simulink model "elsistema"  (R2020b)
settings: Solver=ode15s  StartTime=0.0  StopTime=10  MaxStep=1E-2  RelTol=1e-3
libraries: fl_lib x12, nesl_utility x8, ee_lib x2, pid_lib x1
settings Model: Creator=MSI  LastModifiedBy=hiram
settings SolverCC: AlgebraicLoopSolver=LineSearch
settings DataIOCC: SaveOutput=off  SignalLogging=off  DSMLogging=off  ReturnWorkspaceOutputs=off  TimeSaveName=t
settings DebuggingCC: AlgebraicLoopMsg=none  ArtificialAlgebraicLoopMsg=none  MaxConsecutiveZCsMsg=none  UnconnectedInputMsg=none  UnconnectedOutputMsg=none  UnconnectedLineMsg=none  ModelReferenceExtraNoncontSigs=none  OperatingPointInterfaceChecksumMismatchMsg=none
settings ModelReferenceCC: EnableRefExpFcnMdlSchedulingChecks=off

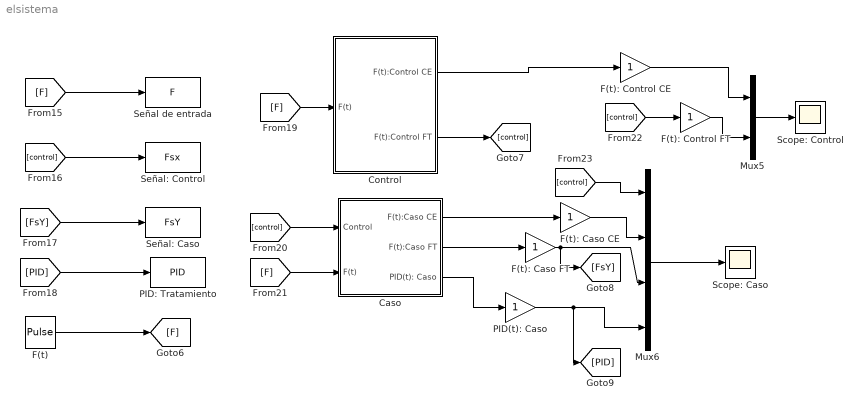
== system elsistema ==
  Caso : Subsystem
  Control : Subsystem
  F(t) : DiscretePulseGenerator  PulseType=Time based  Period=10  PulseWidth=10  PhaseDelay=1
  F(t): Caso CE : Gain
  F(t): Caso FT : Gain
  F(t): Control CE : Gain
  F(t): Control FT : Gain
  Mux5 : Mux  Inputs=2
  Mux6 : Mux
  PID(t): Caso : Gain
  PID: Tratamiento : ToWorkspace  VariableName=PID  SampleTime=-1
  Scope: Caso : Scope
  Scope: Control : Scope
  Señal de entrada : ToWorkspace  VariableName=F  SampleTime=-1
  Señal: Caso : ToWorkspace  VariableName=FsY  SampleTime=-1
  Señal: Control : ToWorkspace  VariableName=Fsx  SampleTime=-1
  wires:
  [F] -> Señal de entrada/1
  [control] -> Señal: Control/1
  [FsY] -> Señal: Caso/1
  [PID] -> PID: Tratamiento/1
  F(t)/1 -> [F]
  [F] -> Control/1(F(t))
  [control] -> Caso/1(Control)
  [F] -> Caso/2(F(t))
  Control/2(F(t):Control FT) -> [control]
  F(t): Control CE/1 -> Mux5/1
  [control] -> F(t): Control FT/1
  F(t): Control FT/1 -> Mux5/2
  Mux5/1 -> Scope: Control/1
  Caso/1(F(t):Caso CE) -> F(t): Caso CE/1
  F(t): Caso CE/1 -> Mux6/2
  [control] -> Mux6/1
  Caso/2(F(t):Caso FT) -> F(t): Caso FT/1
  F(t): Caso FT/1 -> Mux6/3, [FsY]
  PID(t): Caso/1 -> [PID], Mux6/4
  Caso/3(PID(t): Caso) -> PID(t): Caso/1
  Mux6/1 -> Scope: Caso/1
  Control/1(F(t):Control CE) -> F(t): Control CE/1

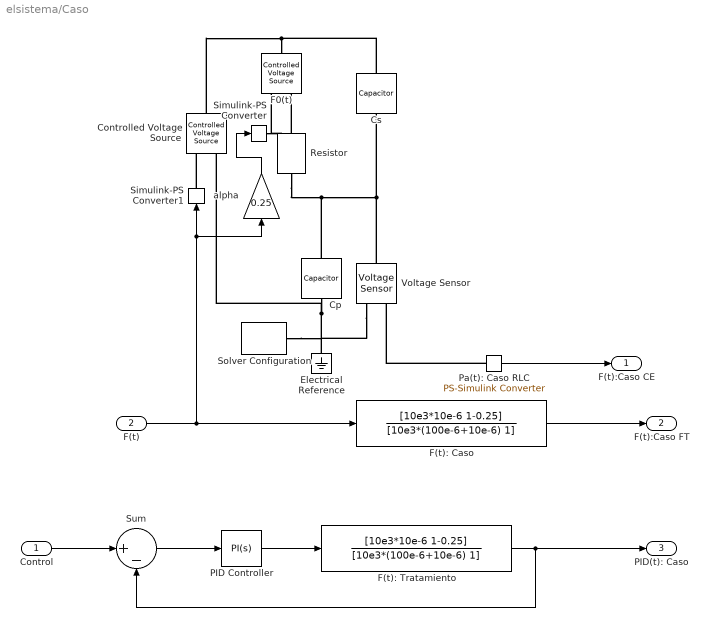
== system elsistema/Caso ==
  Control : Inport
  F(t) : Inport  Port=2
  Controlled Voltage Source : fl_lib/Electrical/Electrical Sources/Controlled Voltage Source
  Cp : fl_lib/Electrical/Electrical Elements/Capacitor  c=1e-6 F  r=1e-6 Ohm  g=0 1/Ohm  i_specify=off  i_priority=None  i=0 A  i_nominal_specify=off  i_nominal_unit=A  i_nominal_value=1  v_specify=off  v_priority=None  v=0 V  v_nominal_specify=off  v_nominal_unit=V  v_nominal_value=1  vc_specify=off  vc_priority=High  vc=0 V  vc_nominal_specify=off  vc_nominal_unit=V  vc_nominal_value=1
  Cs : fl_lib/Electrical/Electrical Elements/Capacitor  c=1e-6 F  r=1e-6 Ohm  g=0 1/Ohm  i_specify=off  i_priority=None  i=0 A  i_nominal_specify=off  i_nominal_unit=A  i_nominal_value=1  v_specify=off  v_priority=None  v=0 V  v_nominal_specify=off  v_nominal_unit=V  v_nominal_value=1  vc_specify=off  vc_priority=High  vc=0 V  vc_nominal_specify=off  vc_nominal_unit=V  vc_nominal_value=1
  Electrical Reference : fl_lib/Electrical/Electrical Elements/Electrical Reference
  F(t): Caso : TransferFcn  Numerator=[10e3*10e-6 1-0.25]  Denominator=[10e3*(100e-6+10e-6) 1]
  F(t): Tratamiento : TransferFcn  Numerator=[10e3*10e-6 1-0.25]  Denominator=[10e3*(100e-6+10e-6) 1]
  F0(t) : fl_lib/Electrical/Electrical Sources/Controlled Voltage Source
  PID Controller : pid_lib/PID Controller  Controller=PI  Form=Parallel  TimeDomain=Continuous-time  UseExternalTs=off  SampleTime=-1  IntegratorMethod=Forward Euler  FilterMethod=Forward Euler  ControllerParametersSource=internal  P=0.21161  I=3765.3621  D=0  UseFilter=on  N=100  TunerSelectOption=Transfer Function Based (PID Tuner App)  InitialConditionSource=internal  InitialConditionForIntegrator=0  InitialConditionForFilter=0  DifferentiatorICPrevScaledInput=0  ExternalReset=none  TrackingMode=off  Kt=1  LimitOutput=off  SatLimitsSource=internal  UpperSaturationLimit=inf  LowerSaturationLimit=-inf  LinearizeAsGain=on  AntiWindupMode=none  Kb=1  POutMin=[]  POutMax=[]  IOutMin=[]  IOutMax=[]  DOutMin=[]  DOutMax=[]  NOutMin=[]  NOutMax=[]  SumOutMin=[]  SumOutMax=[]  SaturationOutMin=[]  SaturationOutMax=[]  PParamMin=[]  PParamMax=[]  IParamMin=[]  IParamMax=[]  DParamMin=[]  DParamMax=[]  NParamMin=[]  NParamMax=[]  KbParamMin=[]  KbParamMax=[]  KtParamMin=[]  KtParamMax=[]  KbOutMin=[]  KbOutMax=[]  KtOutMin=[]  KtOutMax=[]  IntegratorOutMin=[]  IntegratorOutMax=[]  FilterOutMin=[]  FilterOutMax=[]  SumI1OutMin=[]  SumI1OutMax=[]  SumI2OutMin=[]  SumI2OutMax=[]  SumI3OutMin=[]  SumI3OutMax=[]  SumI4OutMin=[]  SumI4OutMax=[]  SumDOutMin=[]  SumDOutMax=[]  DifferentiatorOutMin=[]  DifferentiatorOutMax=[]  FilterDiffOutCoefMin=[]  FilterDiffOutCoefMax=[]  ReciprocalOutMin=[]  ReciprocalOutMax=[]  SumDenOutMin=[]  SumDenOutMax=[]  SumNumOutMin=[]  SumNumOutMax=[]  DivideOutMin=[]  DivideOutMax=[]  UdiffTsProdOutMin=[]  UdiffTsProdOutMax=[]  NTsProdOutMin=[]  NTsProdOutMax=[]  UintegralTsProdOutMin=[]  UintegralTsProdOutMax=[]  UngainTsProdOutMin=[]  UngainTsProdOutMax=[]  IntegratorContinuousStateAttributes=''  IntegratorStateMustResolveToSignalObject=off  IntegratorRTWStateStorageClass=Auto  FilterContinuousStateAttributes=''  FilterStateMustResolveToSignalObject=off  FilterRTWStateStorageClass=Auto  ParallelPVariant=InternalParameters  IdealPVariant=Disabled  IVariant=InternalParameters  DVariant=Disabled  IntegratorVariant=Continuous  SatVariant=Disabled  AWVariant=Passthrough  PCopyVariant=Disabled  TRVariant=Disabled  FdbkBlocksVariant=Forward  IdealPFdbkVariant=Disabled  SatFdbkVariant=Disabled  DerivativeFilterVariant=Disabled  NVariant=Disabled  NCopyVariant=Disabled_SignalSpec  FilterICVariant=Disabled  IntegratorICVariant=InternalICs  ExternalResetVariant=Disabled  TRSumVariant=Passthrough  SumFdbkVariant=Disabled  SumVariant=Sum_PI  TsampFilterVariant=InternalTs  TsampNgainVariant=Passthrough  TsampIntegralVariant=Passthrough  ExternalSaturationOutDataTypeStr=Inherit: Same as second input
  Pa(t): Caso RLC : nesl_utility/PS-Simulink Converter  PhysicalDomain=network_engine_domain  SubClassName=ps_output  LeftPortType=input  RightPortType=output  PseudoPeriodic=off  Frequencies=[]  Unit=inherit  AffineConversion=off
  Resistor : ee_lib/Passive/Resistor  R=1 Ohm  R_tol=5  enable_R_tol=0  tol_distribution=1  nSigma=4  enable_operating_limits=0  operating_limit_action=2  max_working_voltage=100 V  power_rating=1 W  enable_faults=0  fault_action=1  R_faulted=inf Ohm  enable_temporal_fault=0  t_fault=1 s  enable_behavioral_fault=0  max_permissible_current=1 A  t_fail_on_current=1 s  noise_mode=0  sample_time=1e-3 s  repeatability=1  auto_seed=3499211588  user_seed=0  Tdevice=25 degC  alpha=3.93e-3 1/K  Tmeas=25 degC  thermal_mass=100 J/K  power_derating_T1=70 degC  power_derating_T2=155 degC  operating_temperature_range_vec=[-50, 150] degC  temperature_specify=off  temperature_priority=High  temperature=298.15 K  temperature_nominal_specify=off  temperature_nominal_unit=K  temperature_nominal_value=1
  Simulink-PS Converter : nesl_utility/Simulink-PS Converter  PhysicalDomain=network_engine_domain  SubClassName=ps_input  LeftPortType=input  RightPortType=output  PseudoPeriodic=off  Frequencies=[]  NoiseDistribution=none  NoiseParameters=[]  Unit=1  AffineConversion=off  FilteringAndDerivatives=provide  SimscapeFilterOrder=1  InputFilterTimeConstant=0.001  UdotUserProvided=0
  Simulink-PS Converter1 : nesl_utility/Simulink-PS Converter  PhysicalDomain=network_engine_domain  SubClassName=ps_input  LeftPortType=input  RightPortType=output  PseudoPeriodic=off  Frequencies=[]  NoiseDistribution=none  NoiseParameters=[]  Unit=1  AffineConversion=off  FilteringAndDerivatives=provide  SimscapeFilterOrder=1  InputFilterTimeConstant=0.001  UdotUserProvided=0
  Solver Configuration : nesl_utility/Solver Configuration  PhysicalDomain=network_engine_domain  SubClassName=solver  LeftPortType=input  RightPortType=generic  Tones=[]  Harmonics=[]  SimulateNoise=off  Profile=off  UseLocalSampling=off  EnableSwitchedLinearOptims=on  FrequencyDomain=off  UseCCode=off  RelTol=0.001  AbsTol=1e-06  MinStep=1e-09  ToWorkspace=off  RevertToSquareIcSolve=off  NumHomotopyIterations=100  PhasorMode=off  PhasorModeNumHarmonics=1  DoDC=off  ResidualTolerance=1e-09  UseLocalSolver=off  LocalSolverChoice=NE_BACKWARD_EULER_ADVANCER  LocalSolverSampleTime=0.001  DoFixedCost=off  MaxNonlinIter=3  MaxModeIter=2  ComputeImpulses=off  ImpulseIterations=2  LinearAlgebra=auto  EquationFormulation=NE_TIME_EF  DelaysMemoryBudget=1024  AutomaticFiltering=on  FilteringTimeConstant=0.001  PartitionStorageMethod=AS_NEEDED  PartitionMemoryBudget=1024  PartitionMethod=ROBUST
  Sum : Sum  Inputs=|+-
  Voltage Sensor : fl_lib/Electrical/Electrical Sensors/Voltage Sensor
  alpha : Gain  Gain=0.25
  F(t):Caso CE : Outport
  F(t):Caso FT : Outport  Port=2
  PID(t): Caso : Outport  Port=3
  wires:
  alpha/1 -> Simulink-PS Converter/1
  F(t)/1 -> F(t): Caso/1, alpha/1, Simulink-PS Converter1/1
  Pa(t): Caso RLC/1 -> F(t):Caso CE/1
  F(t): Caso/1 -> F(t):Caso FT/1
  Control/1 -> Sum/1
  Sum/1 -> PID Controller/1
  PID Controller/1 -> F(t): Tratamiento/1
  F(t): Tratamiento/1 -> Sum/2, PID(t): Caso/1
  connections:
  Controlled Voltage Source/LConn1 -- Cs/LConn1 -- F0(t)/LConn1
  Resistor/LConn1 -- F0(t)/RConn2
  Resistor/RConn1 -- Cp/LConn1 -- Cs/RConn1 -- Voltage Sensor/LConn1
  Cp/RConn1 -- Solver Configuration/RConn1 -- Voltage Sensor/RConn2 -- Electrical Reference/LConn1 -- Controlled Voltage Source/RConn2
  Simulink-PS Converter/RConn1 -- F0(t)/RConn1
  Simulink-PS Converter1/RConn1 -- Controlled Voltage Source/RConn1
  Pa(t): Caso RLC/LConn1 -- Voltage Sensor/RConn1

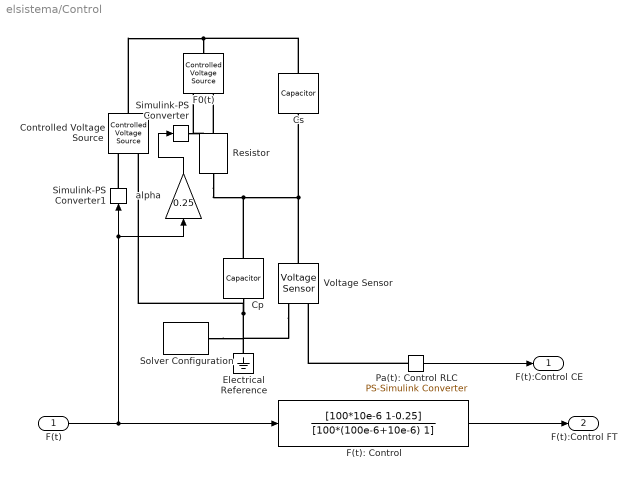
== system elsistema/Control ==
  F(t) : Inport
  Controlled Voltage Source : fl_lib/Electrical/Electrical Sources/Controlled Voltage Source
  Cp : fl_lib/Electrical/Electrical Elements/Capacitor  c=1e-6 F  r=1e-6 Ohm  g=0 1/Ohm  i_specify=off  i_priority=None  i=0 A  i_nominal_specify=off  i_nominal_unit=A  i_nominal_value=1  v_specify=off  v_priority=None  v=0 V  v_nominal_specify=off  v_nominal_unit=V  v_nominal_value=1  vc_specify=off  vc_priority=High  vc=0 V  vc_nominal_specify=off  vc_nominal_unit=V  vc_nominal_value=1
  Cs : fl_lib/Electrical/Electrical Elements/Capacitor  c=1e-6 F  r=1e-6 Ohm  g=0 1/Ohm  i_specify=off  i_priority=None  i=0 A  i_nominal_specify=off  i_nominal_unit=A  i_nominal_value=1  v_specify=off  v_priority=None  v=0 V  v_nominal_specify=off  v_nominal_unit=V  v_nominal_value=1  vc_specify=off  vc_priority=High  vc=0 V  vc_nominal_specify=off  vc_nominal_unit=V  vc_nominal_value=1
  Electrical Reference : fl_lib/Electrical/Electrical Elements/Electrical Reference
  F(t): Control : TransferFcn  Numerator=[100*10e-6 1-0.25]  Denominator=[100*(100e-6+10e-6) 1]
  F0(t) : fl_lib/Electrical/Electrical Sources/Controlled Voltage Source
  Pa(t): Control RLC : nesl_utility/PS-Simulink Converter  PhysicalDomain=network_engine_domain  SubClassName=ps_output  LeftPortType=input  RightPortType=output  PseudoPeriodic=off  Frequencies=[]  Unit=inherit  AffineConversion=off
  Resistor : ee_lib/Passive/Resistor  R=1 Ohm  R_tol=5  enable_R_tol=0  tol_distribution=1  nSigma=4  enable_operating_limits=0  operating_limit_action=2  max_working_voltage=100 V  power_rating=1 W  enable_faults=0  fault_action=1  R_faulted=inf Ohm  enable_temporal_fault=0  t_fault=1 s  enable_behavioral_fault=0  max_permissible_current=1 A  t_fail_on_current=1 s  noise_mode=0  sample_time=1e-3 s  repeatability=1  auto_seed=3499211588  user_seed=0  Tdevice=25 degC  alpha=3.93e-3 1/K  Tmeas=25 degC  thermal_mass=100 J/K  power_derating_T1=70 degC  power_derating_T2=155 degC  operating_temperature_range_vec=[-50, 150] degC  temperature_specify=off  temperature_priority=High  temperature=298.15 K  temperature_nominal_specify=off  temperature_nominal_unit=K  temperature_nominal_value=1
  Simulink-PS Converter : nesl_utility/Simulink-PS Converter  PhysicalDomain=network_engine_domain  SubClassName=ps_input  LeftPortType=input  RightPortType=output  PseudoPeriodic=off  Frequencies=[]  NoiseDistribution=none  NoiseParameters=[]  Unit=1  AffineConversion=off  FilteringAndDerivatives=provide  SimscapeFilterOrder=1  InputFilterTimeConstant=0.001  UdotUserProvided=0
  Simulink-PS Converter1 : nesl_utility/Simulink-PS Converter  PhysicalDomain=network_engine_domain  SubClassName=ps_input  LeftPortType=input  RightPortType=output  PseudoPeriodic=off  Frequencies=[]  NoiseDistribution=none  NoiseParameters=[]  Unit=1  AffineConversion=off  FilteringAndDerivatives=provide  SimscapeFilterOrder=1  InputFilterTimeConstant=0.001  UdotUserProvided=0
  Solver Configuration : nesl_utility/Solver Configuration  PhysicalDomain=network_engine_domain  SubClassName=solver  LeftPortType=input  RightPortType=generic  Tones=[]  Harmonics=[]  SimulateNoise=off  Profile=off  UseLocalSampling=off  EnableSwitchedLinearOptims=on  FrequencyDomain=off  UseCCode=off  RelTol=0.001  AbsTol=1e-06  MinStep=1e-09  ToWorkspace=off  RevertToSquareIcSolve=off  NumHomotopyIterations=100  PhasorMode=off  PhasorModeNumHarmonics=1  DoDC=off  ResidualTolerance=1e-09  UseLocalSolver=off  LocalSolverChoice=NE_BACKWARD_EULER_ADVANCER  LocalSolverSampleTime=0.001  DoFixedCost=off  MaxNonlinIter=3  MaxModeIter=2  ComputeImpulses=off  ImpulseIterations=2  LinearAlgebra=auto  EquationFormulation=NE_TIME_EF  DelaysMemoryBudget=1024  AutomaticFiltering=on  FilteringTimeConstant=0.001  PartitionStorageMethod=AS_NEEDED  PartitionMemoryBudget=1024  PartitionMethod=ROBUST
  Voltage Sensor : fl_lib/Electrical/Electrical Sensors/Voltage Sensor
  alpha : Gain  Gain=0.25
  F(t):Control CE : Outport
  F(t):Control FT : Outport  Port=2
  wires:
  alpha/1 -> Simulink-PS Converter/1
  Pa(t): Control RLC/1 -> F(t):Control CE/1
  F(t): Control/1 -> F(t):Control FT/1
  F(t)/1 -> F(t): Control/1, alpha/1, Simulink-PS Converter1/1
  connections:
  Resistor/RConn1 -- Cp/LConn1 -- Cs/RConn1 -- Voltage Sensor/LConn1
  Cp/RConn1 -- Solver Configuration/RConn1 -- Voltage Sensor/RConn2 -- Electrical Reference/LConn1 -- Controlled Voltage Source/RConn2
  Controlled Voltage Source/LConn1 -- Cs/LConn1 -- F0(t)/LConn1
  Resistor/LConn1 -- F0(t)/RConn2
  Simulink-PS Converter1/RConn1 -- Controlled Voltage Source/RConn1
  Simulink-PS Converter/RConn1 -- F0(t)/RConn1
  Pa(t): Control RLC/LConn1 -- Voltage Sensor/RConn1
